simulink model "Battery_model"  (R2025a)
settings: Solver=VariableStepAuto  StartTime=0.0  StopTime=1369  RelTol=1e-3
undefined symbols (not defined in the file): batt
settings Model: Creator=deepakkumarn  LastModifiedBy=deepakkumarn

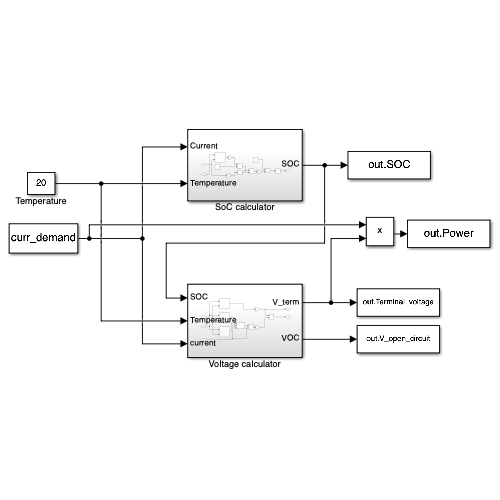
[thumbnail: Simulink's stored preview of the top-level diagram]
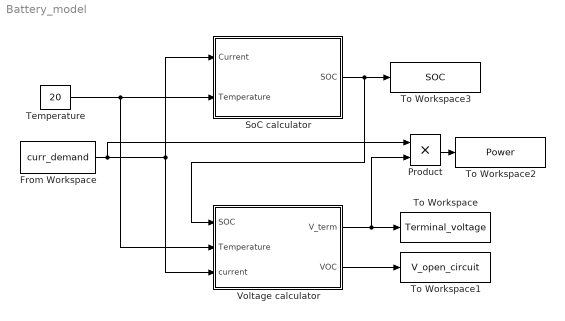
== system Battery_model ==
  From Workspace : FromWorkspace  VariableName=curr_demand
  Product : Product
  SoC calculator : Subsystem
  Temperature : Constant  Value=20
  To Workspace : ToWorkspace  VariableName=Terminal_voltage  SaveFormat=Timeseries  SampleTime=-1
  To Workspace1 : ToWorkspace  VariableName=V_open_circuit  SaveFormat=Timeseries  SampleTime=-1
  To Workspace2 : ToWorkspace  VariableName=Power  SaveFormat=Timeseries  SampleTime=-1
  To Workspace3 : ToWorkspace  VariableName=SOC  SaveFormat=Timeseries  SampleTime=-1
  Voltage calculator : Subsystem
  wires:
  From Workspace/1 -> Product/1, Voltage calculator/3(current), SoC calculator/1(Current)
  Temperature/1 -> Voltage calculator/2(Temperature), SoC calculator/2(Temperature)
  SoC calculator/1(SOC) -> Voltage calculator/1(SOC), To Workspace3/1
  Voltage calculator/2(VOC) -> To Workspace1/1
  Voltage calculator/1(V_term) -> Product/2, To Workspace/1
  Product/1 -> To Workspace2/1

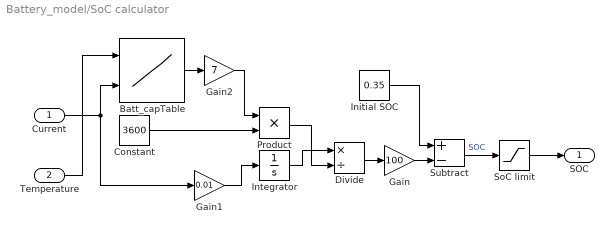
== system Battery_model/SoC calculator ==
  Current : Inport
  Temperature : Inport  Port=2
  Batt_capTable : Lookup_n-D  BreakpointsForDimension1=batt.cap_max.temp  BreakpointsForDimension2=batt.cap_max.curr  Table=batt.cap_max.cap_max  InternalRulePriority=Speed  RndMeth=Simplest
      settings: InputPortMap=u0,u1
  Constant : Constant  Value=3600
  Divide : Product  Inputs=*/
  Gain : Gain  Gain=100
  Gain1 : Gain  Gain=0.01
  Gain2 : Gain  Gain=7
  Initial SOC : Constant  Value=0.35
  Integrator : Integrator
  Product : Product
  SoC limit : Saturate  UpperLimit=0.92  LowerLimit=0.28
  Subtract : Sum  Inputs=+-
  SOC : Outport
  wires:
  Batt_capTable/1 -> Gain2/1
  Temperature/1 -> Batt_capTable/1
  Constant/1 -> Product/2
  Product/1 -> Divide/2
  Current/1 -> Gain1/1, Batt_capTable/2
  Initial SOC/1 -> Subtract/1
  Divide/1 -> Gain/1
  Subtract/1 -> SoC limit/1  "SOC"
  Integrator/1 -> Divide/1
  Gain/1 -> Subtract/2
  SoC limit/1 -> SOC/1
  Gain1/1 -> Integrator/1
  Gain2/1 -> Product/1

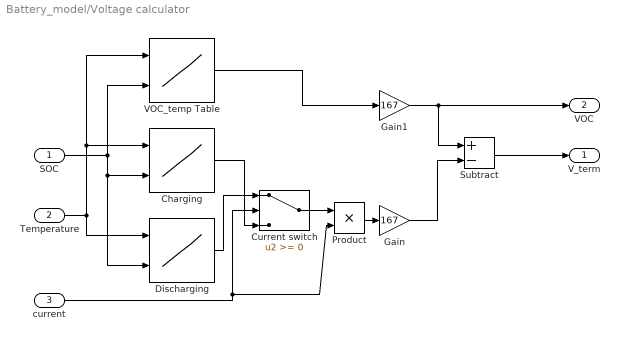
== system Battery_model/Voltage calculator ==
  SOC : Inport
  Temperature : Inport  Port=2
  current : Inport  Port=3
  Charging : Lookup_n-D  BreakpointsForDimension1=batt.r_int_chg.temp  BreakpointsForDimension2=batt.r_int_chg.soc  Table=batt.r_int_chg.r_int  InternalRulePriority=Speed  RndMeth=Simplest
      settings: InputPortMap=u0,u1
  Current switch : Switch  SaturateOnIntegerOverflow=off  InputSameDT=off
  Discharging : Lookup_n-D  BreakpointsForDimension1=batt.r_int_dis.temp  BreakpointsForDimension2=batt.r_int_dis.soc  Table=batt.r_int_dis.r_int  InternalRulePriority=Speed  RndMeth=Simplest
      settings: InputPortMap=u0,u1
  Gain : Gain  Gain=167
  Gain1 : Gain  Gain=167
  Product : Product
  Subtract : Sum  Inputs=+-
  VOC_temp Table : Lookup_n-D  BreakpointsForDimension1=batt.voc.temp  BreakpointsForDimension2=batt.voc.soc  Table=batt.voc.voc  InternalRulePriority=Speed  RndMeth=Simplest
      settings: InputPortMap=u0,u1
  V_term : Outport
  VOC : Outport  Port=2
  wires:
  current/1 -> Product/2, Current switch/2
  SOC/1 -> VOC_temp Table/2, Charging/2, Discharging/2
  Temperature/1 -> Discharging/1, VOC_temp Table/1, Charging/1
  Charging/1 -> Current switch/3
  Discharging/1 -> Current switch/1
  Current switch/1 -> Product/1
  VOC_temp Table/1 -> Gain1/1
  Product/1 -> Gain/1
  Subtract/1 -> V_term/1
  Gain/1 -> Subtract/2
  Gain1/1 -> VOC/1, Subtract/1
